simulink library "SCR"  (R2024b)
settings: Solver=VariableStepAuto  StartTime=0.0  StopTime=10.0  RelTol=1e-3
libraries: nesl_utility x29, fl_lib x26, sm_lib x16, ee_lib x7, slpidlib x4
(part 1 of 2)
settings Model: Creator=Michael  LastModifiedBy=Michael

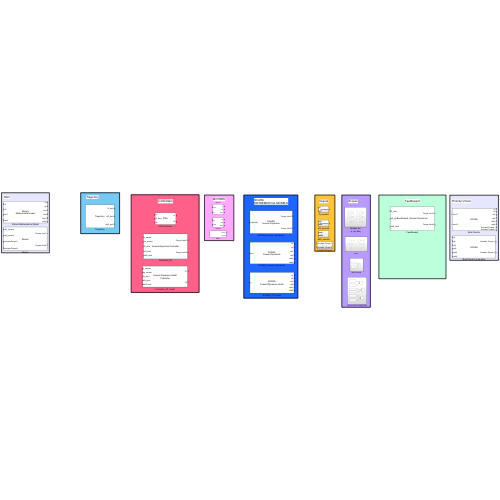
[thumbnail: Simulink's stored preview of the top-level diagram]
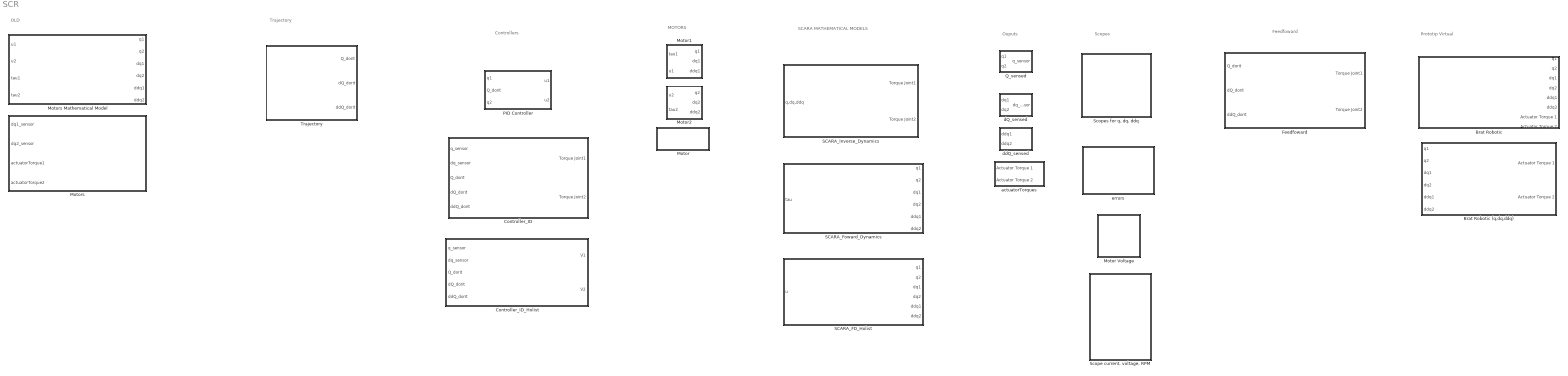
== system SCR ==
  note: MOTORS
  note: SCARA
      | MATHEMATICAL MODELS
  note: Scopes
  note: Ouputs
  note: Trajectory
  note: Controllers
  note: Feedfoward
  note: OLD
  note: Prototip Virtual
  Brat Robotic : Subsystem
      mask Display: disp("SCARA")
  Brat Robotic (q,dq,ddq) : Subsystem
      mask Display: disp("SCARA")
  Controller_ID : Subsystem
      mask Display: disp("Inverse Dynamics Controller")
  Controller_ID_Holist : Subsystem
      mask Display:
      | disp("Inverse Dynamics Holist\n")
      | disp("\nController")
  Feedfoward : Subsystem
      mask Display: disp("Feedfoward (Inverse Dynamics)")
  Motor : Subsystem
  Motor Voltage : Subsystem
  Motor1 : Subsystem
  Motor2 : Subsystem
  Motors : Subsystem
      mask Display: disp("Motors")
  Motors Mathematical Model : Subsystem
      mask Display:
      | disp("Motors\n")
      | disp("\nMathematical model")
  PID Controller : Subsystem
      mask Display: disp("PIDs")
  Q_sensed : Subsystem
  SCARA_FD_Holist : Subsystem
      mask Display:
      | disp("SCARA\n")
      | disp("\nFoward Dynamics Holist")
  SCARA_Foward_Dynamics : Subsystem
      mask Display:
      | disp("SCARA\n")
      | disp("\nFoward Dynamics")
  SCARA_Inverse_Dynamics : Subsystem
      mask Display:
      | disp("SCARA\n")
      | disp("\nInverse Dynamics")
  "Scope current, voltage, RPM" : Subsystem
  "Scopes for q, dq, ddq" : Subsystem
  Trajectory : Subsystem
      mask Display: disp("Trajectory")
  actuatorTorques : Subsystem
  dQ_sensed : Subsystem
  ddQ_sensed : Subsystem
  errors : Subsystem

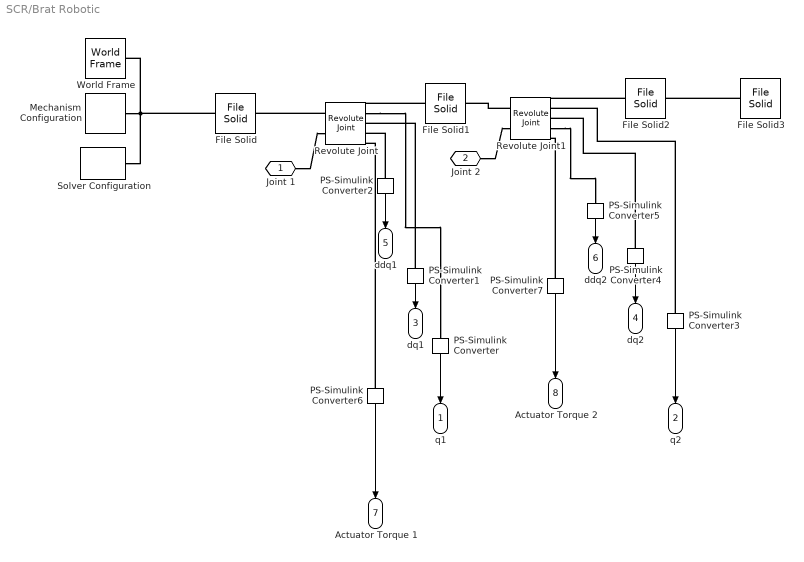
== system SCR/Brat Robotic ==
  File Solid : sm_lib/Body Elements/File Solid  ExtGeomFileName=C:\Users\Michael\Documents\Facultate\AN-IV\SCR\SCARA\robotCAD\baza.step  UnitType=FromFile  ExtGeomFileUnits=m  StepReaderType=HEX  ExportConvexHullGeometry=off  InertiaType=CalculateFromGeometry  BasedOnType=Density  Density=2700  DensityUnits=kg/m^3  Mass=1  MassUnits=kg  CenterOfMass=[0 0 0]  CenterOfMassUnits=m  MomentsOfInertia=[1 1 1]  MomentsOfInertiaUnits=kg*m^2  ProductsOfInertia=[0 0 0]  ProductsOfInertiaUnits=kg*m^2  GraphicType=FromGeometry  MarkerShape=Sphere  MarkerSize=10  GraphicVisPropType=SimpleVisualProperties  GraphicDiffuseColor=[0.5 0.5 0.5]  GraphicOpacity=1  GraphicSpecularColor=[0.5 0.5 0.5 1.0]  GraphicAmbientColor=[0.15 0.15 0.15 1.0]  GraphicEmissiveColor=[0.0 0.0 0.0 1.0]  GraphicShininess=75  DoExposeReferenceFrame=on  SerializedFrames=<Frames><Frame><Id>Frame1</Id><Value><Name>F1</Name><Origin><Source>GeometricFeature</Source><FeatureName>planar surface 2</FeatureName></Origin><PrimaryAxis><DefinedDirection>+Z</DefinedDirection><Source>ReferenceFrame</Source><SourceDirection>+Z</SourceDirection><FeatureName></FeatureName></PrimaryAxis><SecondaryAxis><DefinedDirection>+X</DefinedDirection><Source>ReferenceFrame</Source><SourceDirection>+X</SourceDirection><FeatureName></FeatureName></SecondaryAxis></Value></Frame></Frames>
  File Solid1 : sm_lib/Body Elements/File Solid  ExtGeomFileName=C:\Users\Michael\Documents\Facultate\AN-IV\SCR\SCARA\robotCAD\link1.step  UnitType=FromFile  ExtGeomFileUnits=m  StepReaderType=HEX  ExportConvexHullGeometry=off  InertiaType=CalculateFromGeometry  BasedOnType=Density  Density=2700  DensityUnits=kg/m^3  Mass=1  MassUnits=kg  CenterOfMass=[0 0 0]  CenterOfMassUnits=m  MomentsOfInertia=[1 1 1]  MomentsOfInertiaUnits=kg*m^2  ProductsOfInertia=[0 0 0]  ProductsOfInertiaUnits=kg*m^2  GraphicType=FromGeometry  MarkerShape=Sphere  MarkerSize=10  GraphicVisPropType=SimpleVisualProperties  GraphicDiffuseColor=[0.5 0.5 0.5]  GraphicOpacity=1  GraphicSpecularColor=[0.5 0.5 0.5 1.0]  GraphicAmbientColor=[0.15 0.15 0.15 1.0]  GraphicEmissiveColor=[0.0 0.0 0.0 1.0]  GraphicShininess=75  DoExposeReferenceFrame=on  SerializedFrames=<Frames><Frame><Id>Frame1</Id><Value><Name>F1</Name><Origin><Source>GeometricFeature</Source><FeatureName>circular curve 1</FeatureName></Origin><PrimaryAxis><DefinedDirection>+Z</DefinedDirection><Source>ReferenceFrame</Source><SourceDirection>+Z</SourceDirection><FeatureName></FeatureName></PrimaryAxis><SecondaryAxis><DefinedDirection>+X</DefinedDirection><Source>ReferenceFrame</Source><SourceDirection>+X</SourceDirection><FeatureName></FeatureName></SecondaryAxis></Value></Frame></Frames>
  File Solid2 : sm_lib/Body Elements/File Solid  ExtGeomFileName=C:\Users\Michael\Documents\Facultate\AN-IV\SCR\SCARA\robotCAD\link2.step  UnitType=FromFile  ExtGeomFileUnits=m  StepReaderType=HEX  ExportConvexHullGeometry=off  InertiaType=CalculateFromGeometry  BasedOnType=Density  Density=2700  DensityUnits=kg/m^3  Mass=1  MassUnits=kg  CenterOfMass=[0 0 0]  CenterOfMassUnits=m  MomentsOfInertia=[1 1 1]  MomentsOfInertiaUnits=kg*m^2  ProductsOfInertia=[0 0 0]  ProductsOfInertiaUnits=kg*m^2  GraphicType=FromGeometry  MarkerShape=Sphere  MarkerSize=10  GraphicVisPropType=SimpleVisualProperties  GraphicDiffuseColor=[0.5 0.5 0.5]  GraphicOpacity=1  GraphicSpecularColor=[0.5 0.5 0.5 1.0]  GraphicAmbientColor=[0.15 0.15 0.15 1.0]  GraphicEmissiveColor=[0.0 0.0 0.0 1.0]  GraphicShininess=75  DoExposeReferenceFrame=on  SerializedFrames=<Frames><Frame><Id>Frame1</Id><Value><Name>F1</Name><Origin><Source>GeometricFeature</Source><FeatureName>circular curve 1</FeatureName></Origin><PrimaryAxis><DefinedDirection>+Z</DefinedDirection><Source>ReferenceFrame</Source><SourceDirection>+Z</SourceDirection><FeatureName></FeatureName></PrimaryAxis><SecondaryAxis><DefinedDirection>+X</DefinedDirection><Source>ReferenceFrame</Source><SourceDirection>+X</SourceDirection><FeatureName></FeatureName></SecondaryAxis></Value></Frame></Frames>
  File Solid3 : sm_lib/Body Elements/File Solid  ExtGeomFileName=C:\Users\Michael\Documents\Facultate\AN-IV\SCR\SCARA\robotCAD\efector.step  UnitType=FromFile  ExtGeomFileUnits=m  StepReaderType=HEX  ExportConvexHullGeometry=off  InertiaType=CalculateFromGeometry  BasedOnType=Density  Density=2700  DensityUnits=kg/m^3  Mass=1  MassUnits=kg  CenterOfMass=[0 0 0]  CenterOfMassUnits=m  MomentsOfInertia=[1 1 1]  MomentsOfInertiaUnits=kg*m^2  ProductsOfInertia=[0 0 0]  ProductsOfInertiaUnits=kg*m^2  GraphicType=FromGeometry  MarkerShape=Sphere  MarkerSize=10  GraphicVisPropType=SimpleVisualProperties  GraphicDiffuseColor=[0.5 0.5 0.5]  GraphicOpacity=1  GraphicSpecularColor=[0.5 0.5 0.5 1.0]  GraphicAmbientColor=[0.15 0.15 0.15 1.0]  GraphicEmissiveColor=[0.0 0.0 0.0 1.0]  GraphicShininess=75  DoExposeReferenceFrame=off  SerializedFrames=<Frames><Frame><Id>Frame1</Id><Value><Name>F1</Name><Origin><Source>GeometricFeature</Source><FeatureName>planar surface 1</FeatureName></Origin><PrimaryAxis><DefinedDirection>+Z</DefinedDirection><Source>ReferenceFrame</Source><SourceDirection>+Z</SourceDirection><FeatureName></FeatureName></PrimaryAxis><SecondaryAxis><DefinedDirection>+X</DefinedDirection><Source>ReferenceFrame</Source><SourceDirection>+X</SourceDirection><FeatureName></FeatureName></SecondaryAxis></Value></Frame></Frames>
  Mechanism Configuration : sm_lib/Utilities/Mechanism Configuration  UniformGravity=Constant  GravityVector=[0 0 -9.80665]  GravityVectorUnits=m/s^2  LinearizationDelta=0.001  JointModeTransitionNonlinearIterations=2
  PS-Simulink Converter{,2..3,5..7} (6 alike) : nesl_utility/PS-Simulink Converter  PhysicalDomain=network_engine_domain  SubClassName=ps_output  LeftPortType=input  RightPortType=output  PseudoPeriodic=off  Frequencies=[]  VectorFormat=inherit  Unit=inherit  AffineConversion=off
  PS-Simulink Converter1 : nesl_utility/PS-Simulink Converter  PhysicalDomain=network_engine_domain  SubClassName=ps_output  LeftPortType=input  RightPortType=output  PseudoPeriodic=off  Frequencies=[]  VectorFormat=inherit  Unit=rad/s  AffineConversion=off
  PS-Simulink Converter4 : nesl_utility/PS-Simulink Converter  PhysicalDomain=network_engine_domain  SubClassName=ps_output  LeftPortType=input  RightPortType=output  PseudoPeriodic=off  Frequencies=[]  VectorFormat=inherit  Unit=rad/s  AffineConversion=off
  Revolute Joint : sm_lib/Joints/Revolute Joint  JointMode=Normal  CompositeWrenchDir=FollowerOnBase  CompositeWrenchFrame=BaseFrame  SenseConstraintForce=off  SenseConstraintTorque=off  SenseTotalForce=off  SenseTotalTorque=off  PositionTargetSpecify=off  PositionTargetPriority=High  PositionTargetValue=0  PositionTargetValueUnits=deg  VelocityTargetSpecify=off  VelocityTargetPriority=High  VelocityTargetValue=0  VelocityTargetValueUnits=deg/s  EquilibriumPosition=0  EquilibriumPositionUnits=deg  SpringStiffness=0  SpringStiffnessUnits=N*m/deg  DampingCoefficient=0  DampingCoefficientUnits=N*m/(deg/s)  LowerLimitSpecify=off  LowerLimitBound=-90  LowerLimitBoundUnits=deg  LowerLimitStiffness=1e4  LowerLimitStiffnessUnits=N*m/deg  LowerLimitDamping=10  LowerLimitDampingUnits=N*m/(deg/s)  LowerLimitTransitionRegionWidth=0.1  LowerLimitTransitionRegionWidthUnits=deg  UpperLimitSpecify=off  UpperLimitBound=90  UpperLimitBoundUnits=deg  UpperLimitStiffness=1e4  UpperLimitStiffnessUnits=N*m/deg  UpperLimitDamping=10  UpperLimitDampingUnits=N*m/(deg/s)  UpperLimitTransitionRegionWidth=0.1  UpperLimitTransitionRegionWidthUnits=deg  TorqueActuationMode=InputTorque  MotionActuationMode=ComputedMotion  SensePosition=on  SenseVelocity=on  SenseAcceleration=on  SenseTorqueForce=on  SenseLowerLimitTorqueForce=off  SenseUpperLimitTorqueForce=off
  Revolute Joint1 : sm_lib/Joints/Revolute Joint  JointMode=Normal  CompositeWrenchDir=FollowerOnBase  CompositeWrenchFrame=BaseFrame  SenseConstraintForce=off  SenseConstraintTorque=off  SenseTotalForce=off  SenseTotalTorque=off  PositionTargetSpecify=off  PositionTargetPriority=High  PositionTargetValue=0  PositionTargetValueUnits=deg  VelocityTargetSpecify=off  VelocityTargetPriority=High  VelocityTargetValue=0  VelocityTargetValueUnits=deg/s  EquilibriumPosition=0  EquilibriumPositionUnits=deg  SpringStiffness=0  SpringStiffnessUnits=N*m/deg  DampingCoefficient=0  DampingCoefficientUnits=N*m/(deg/s)  LowerLimitSpecify=off  LowerLimitBound=-90  LowerLimitBoundUnits=deg  LowerLimitStiffness=1e4  LowerLimitStiffnessUnits=N*m/deg  LowerLimitDamping=10  LowerLimitDampingUnits=N*m/(deg/s)  LowerLimitTransitionRegionWidth=0.1  LowerLimitTransitionRegionWidthUnits=deg  UpperLimitSpecify=off  UpperLimitBound=90  UpperLimitBoundUnits=deg  UpperLimitStiffness=1e4  UpperLimitStiffnessUnits=N*m/deg  UpperLimitDamping=10  UpperLimitDampingUnits=N*m/(deg/s)  UpperLimitTransitionRegionWidth=0.1  UpperLimitTransitionRegionWidthUnits=deg  TorqueActuationMode=InputTorque  MotionActuationMode=ComputedMotion  SensePosition=on  SenseVelocity=on  SenseAcceleration=on  SenseTorqueForce=on  SenseLowerLimitTorqueForce=off  SenseUpperLimitTorqueForce=off
  Solver Configuration : nesl_utility/Solver Configuration  PhysicalDomain=network_engine_domain  SubClassName=solver  LeftPortType=input  RightPortType=generic  Tones=[]  Harmonics=[]  SimulateNoise=off  Profile=off  UseLocalSampling=off  EnableSwitchedLinearOptims=on  FrequencyDomain=off  UseCCode=off  RelTol=0.001  AbsTol=0.001  MinStep=1e-09  ToWorkspace=off  RevertToSquareIcSolve=off  NumHomotopyIterations=100  PhasorMode=off  PhasorModeNumHarmonics=1  ConsistencySolver=NEWTON_XTOL_AFTER_FTOL  IndexReductionMethod=DerivativeReplacement  DoDC=off  ResidualTolerance=1e-09  ConsistencyTolSource=GLOBAL  ConsistencyAbsTol=0.001  ConsistencyRelTol=0.001  ConsistencyTolFactor=0.001  UseLocalSolver=off  LocalSolverChoice=NE_BACKWARD_EULER_ADVANCER  ResolveIndetEquations=on  FunctionEvalNumThread=1  LocalSolverSampleTime=0.001  DoFixedCost=off  MaxNonlinIter=3  MaxModeIter=2  ComputeImpulses=off  ImpulseIterations=2  LinearAlgebra=auto  LinearAlgebraNumThread=0  EquationFormulation=NE_TIME_EF  DelaysMemoryBudget=1024  AutomaticFiltering=on  FilteringTimeConstant=0.001  PartitionStorageMethod=AS_NEEDED  PartitionMemoryBudget=1024  PartitionMethod=ROBUST  MultibodyUseLocalSolver=off  MultibodyLocalSolverChoice=ODE1  MultibodyLocalSolverSampleTime=0.001
  World Frame : sm_lib/Frames and Transforms/World Frame
  Joint 1 : PMIOPort  Side=Left
  Joint 2 : PMIOPort  Port=2  Side=Left
  q1 : Outport
  q2 : Outport  Port=2
  dq1 : Outport  Port=3
  dq2 : Outport  Port=4
  ddq1 : Outport  Port=5
  ddq2 : Outport  Port=6
  Actuator Torque 1 : Outport  Port=7
  Actuator Torque 2 : Outport  Port=8
  wires:
  PS-Simulink Converter2/1 -> ddq1/1
  PS-Simulink Converter1/1 -> dq1/1
  PS-Simulink Converter/1 -> q1/1
  PS-Simulink Converter5/1 -> ddq2/1
  PS-Simulink Converter4/1 -> dq2/1
  PS-Simulink Converter3/1 -> q2/1
  PS-Simulink Converter6/1 -> Actuator Torque 1/1
  PS-Simulink Converter7/1 -> Actuator Torque 2/1
  connections:
  File Solid/RConn1 -- Mechanism Configuration/RConn1 -- Solver Configuration/RConn1 -- World Frame/RConn1
  Revolute Joint/LConn1 -- File Solid/LConn1
  File Solid1/RConn1 -- Revolute Joint/RConn1
  Revolute Joint1/LConn1 -- File Solid1/LConn1
  File Solid2/RConn1 -- Revolute Joint1/RConn1
  File Solid3/LConn1 -- File Solid2/LConn1
  Joint 1/RConn1 -- Revolute Joint/LConn2
  Joint 2/RConn1 -- Revolute Joint1/LConn2
  Revolute Joint/RConn2 -- PS-Simulink Converter/LConn1
  PS-Simulink Converter1/LConn1 -- Revolute Joint/RConn3
  PS-Simulink Converter2/LConn1 -- Revolute Joint/RConn4
  Revolute Joint1/RConn4 -- PS-Simulink Converter5/LConn1
  PS-Simulink Converter4/LConn1 -- Revolute Joint1/RConn3
  PS-Simulink Converter3/LConn1 -- Revolute Joint1/RConn2
  PS-Simulink Converter6/LConn1 -- Revolute Joint/RConn5
  PS-Simulink Converter7/LConn1 -- Revolute Joint1/RConn5

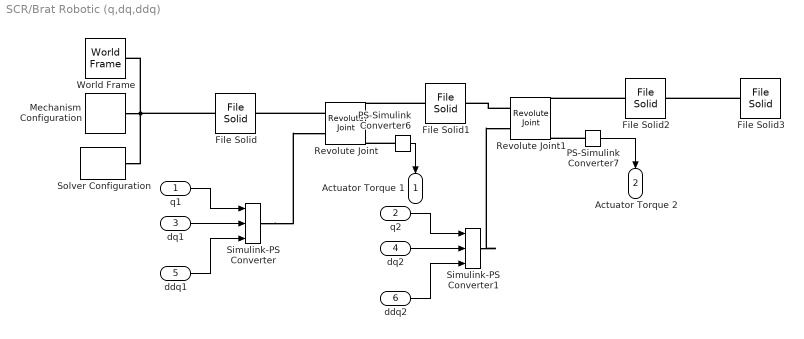
== system SCR/Brat Robotic (q,dq,ddq) ==
  q1 : Inport
  q2 : Inport  Port=2
  dq1 : Inport  Port=3
  dq2 : Inport  Port=4
  ddq1 : Inport  Port=5
  ddq2 : Inport  Port=6
  File Solid : sm_lib/Body Elements/File Solid  ExtGeomFileName=C:\Users\Michael\Documents\Facultate\AN-IV\SCR\SCARA\robotCAD\baza.step  UnitType=FromFile  ExtGeomFileUnits=m  StepReaderType=HEX  ExportConvexHullGeometry=off  InertiaType=CalculateFromGeometry  BasedOnType=Density  Density=2700  DensityUnits=kg/m^3  Mass=1  MassUnits=kg  CenterOfMass=[0 0 0]  CenterOfMassUnits=m  MomentsOfInertia=[1 1 1]  MomentsOfInertiaUnits=kg*m^2  ProductsOfInertia=[0 0 0]  ProductsOfInertiaUnits=kg*m^2  GraphicType=FromGeometry  MarkerShape=Sphere  MarkerSize=10  GraphicVisPropType=SimpleVisualProperties  GraphicDiffuseColor=[0.5 0.5 0.5]  GraphicOpacity=1  GraphicSpecularColor=[0.5 0.5 0.5 1.0]  GraphicAmbientColor=[0.15 0.15 0.15 1.0]  GraphicEmissiveColor=[0.0 0.0 0.0 1.0]  GraphicShininess=75  DoExposeReferenceFrame=on  SerializedFrames=<Frames><Frame><Id>Frame1</Id><Value><Name>F1</Name><Origin><Source>GeometricFeature</Source><FeatureName>planar surface 2</FeatureName></Origin><PrimaryAxis><DefinedDirection>+Z</DefinedDirection><Source>ReferenceFrame</Source><SourceDirection>+Z</SourceDirection><FeatureName></FeatureName></PrimaryAxis><SecondaryAxis><DefinedDirection>+X</DefinedDirection><Source>ReferenceFrame</Source><SourceDirection>+X</SourceDirection><FeatureName></FeatureName></SecondaryAxis></Value></Frame></Frames>
  File Solid1 : sm_lib/Body Elements/File Solid  ExtGeomFileName=C:\Users\Michael\Documents\Facultate\AN-IV\SCR\SCARA\robotCAD\link1.step  UnitType=FromFile  ExtGeomFileUnits=m  StepReaderType=HEX  ExportConvexHullGeometry=off  InertiaType=CalculateFromGeometry  BasedOnType=Density  Density=2700  DensityUnits=kg/m^3  Mass=1  MassUnits=kg  CenterOfMass=[0 0 0]  CenterOfMassUnits=m  MomentsOfInertia=[1 1 1]  MomentsOfInertiaUnits=kg*m^2  ProductsOfInertia=[0 0 0]  ProductsOfInertiaUnits=kg*m^2  GraphicType=FromGeometry  MarkerShape=Sphere  MarkerSize=10  GraphicVisPropType=SimpleVisualProperties  GraphicDiffuseColor=[0.5 0.5 0.5]  GraphicOpacity=1  GraphicSpecularColor=[0.5 0.5 0.5 1.0]  GraphicAmbientColor=[0.15 0.15 0.15 1.0]  GraphicEmissiveColor=[0.0 0.0 0.0 1.0]  GraphicShininess=75  DoExposeReferenceFrame=on  SerializedFrames=<Frames><Frame><Id>Frame1</Id><Value><Name>F1</Name><Origin><Source>GeometricFeature</Source><FeatureName>circular curve 1</FeatureName></Origin><PrimaryAxis><DefinedDirection>+Z</DefinedDirection><Source>ReferenceFrame</Source><SourceDirection>+Z</SourceDirection><FeatureName></FeatureName></PrimaryAxis><SecondaryAxis><DefinedDirection>+X</DefinedDirection><Source>ReferenceFrame</Source><SourceDirection>+X</SourceDirection><FeatureName></FeatureName></SecondaryAxis></Value></Frame></Frames>
  File Solid2 : sm_lib/Body Elements/File Solid  ExtGeomFileName=C:\Users\Michael\Documents\Facultate\AN-IV\SCR\SCARA\robotCAD\link2.step  UnitType=FromFile  ExtGeomFileUnits=m  StepReaderType=HEX  ExportConvexHullGeometry=off  InertiaType=CalculateFromGeometry  BasedOnType=Density  Density=2700  DensityUnits=kg/m^3  Mass=1  MassUnits=kg  CenterOfMass=[0 0 0]  CenterOfMassUnits=m  MomentsOfInertia=[1 1 1]  MomentsOfInertiaUnits=kg*m^2  ProductsOfInertia=[0 0 0]  ProductsOfInertiaUnits=kg*m^2  GraphicType=FromGeometry  MarkerShape=Sphere  MarkerSize=10  GraphicVisPropType=SimpleVisualProperties  GraphicDiffuseColor=[0.5 0.5 0.5]  GraphicOpacity=1  GraphicSpecularColor=[0.5 0.5 0.5 1.0]  GraphicAmbientColor=[0.15 0.15 0.15 1.0]  GraphicEmissiveColor=[0.0 0.0 0.0 1.0]  GraphicShininess=75  DoExposeReferenceFrame=on  SerializedFrames=<Frames><Frame><Id>Frame1</Id><Value><Name>F1</Name><Origin><Source>GeometricFeature</Source><FeatureName>circular curve 1</FeatureName></Origin><PrimaryAxis><DefinedDirection>+Z</DefinedDirection><Source>ReferenceFrame</Source><SourceDirection>+Z</SourceDirection><FeatureName></FeatureName></PrimaryAxis><SecondaryAxis><DefinedDirection>+X</DefinedDirection><Source>ReferenceFrame</Source><SourceDirection>+X</SourceDirection><FeatureName></FeatureName></SecondaryAxis></Value></Frame></Frames>
  File Solid3 : sm_lib/Body Elements/File Solid  ExtGeomFileName=C:\Users\Michael\Documents\Facultate\AN-IV\SCR\SCARA\robotCAD\efector.step  UnitType=FromFile  ExtGeomFileUnits=m  StepReaderType=HEX  ExportConvexHullGeometry=off  InertiaType=CalculateFromGeometry  BasedOnType=Density  Density=2700  DensityUnits=kg/m^3  Mass=1  MassUnits=kg  CenterOfMass=[0 0 0]  CenterOfMassUnits=m  MomentsOfInertia=[1 1 1]  MomentsOfInertiaUnits=kg*m^2  ProductsOfInertia=[0 0 0]  ProductsOfInertiaUnits=kg*m^2  GraphicType=FromGeometry  MarkerShape=Sphere  MarkerSize=10  GraphicVisPropType=SimpleVisualProperties  GraphicDiffuseColor=[0.5 0.5 0.5]  GraphicOpacity=1  GraphicSpecularColor=[0.5 0.5 0.5 1.0]  GraphicAmbientColor=[0.15 0.15 0.15 1.0]  GraphicEmissiveColor=[0.0 0.0 0.0 1.0]  GraphicShininess=75  DoExposeReferenceFrame=off  SerializedFrames=<Frames><Frame><Id>Frame1</Id><Value><Name>F1</Name><Origin><Source>GeometricFeature</Source><FeatureName>planar surface 1</FeatureName></Origin><PrimaryAxis><DefinedDirection>+Z</DefinedDirection><Source>ReferenceFrame</Source><SourceDirection>+Z</SourceDirection><FeatureName></FeatureName></PrimaryAxis><SecondaryAxis><DefinedDirection>+X</DefinedDirection><Source>ReferenceFrame</Source><SourceDirection>+X</SourceDirection><FeatureName></FeatureName></SecondaryAxis></Value></Frame></Frames>
  Mechanism Configuration : sm_lib/Utilities/Mechanism Configuration  UniformGravity=Constant  GravityVector=[0 0 -9.80665]  GravityVectorUnits=m/s^2  LinearizationDelta=0.001  JointModeTransitionNonlinearIterations=2
  PS-Simulink Converter6 : nesl_utility/PS-Simulink Converter  PhysicalDomain=network_engine_domain  SubClassName=ps_output  LeftPortType=input  RightPortType=output  PseudoPeriodic=off  Frequencies=[]  VectorFormat=inherit  Unit=inherit  AffineConversion=off
  PS-Simulink Converter7 : nesl_utility/PS-Simulink Converter  PhysicalDomain=network_engine_domain  SubClassName=ps_output  LeftPortType=input  RightPortType=output  PseudoPeriodic=off  Frequencies=[]  VectorFormat=inherit  Unit=inherit  AffineConversion=off
  Revolute Joint : sm_lib/Joints/Revolute Joint  JointMode=Normal  CompositeWrenchDir=FollowerOnBase  CompositeWrenchFrame=BaseFrame  SenseConstraintForce=off  SenseConstraintTorque=off  SenseTotalForce=off  SenseTotalTorque=off  PositionTargetSpecify=off  PositionTargetPriority=High  PositionTargetValue=0  PositionTargetValueUnits=deg  VelocityTargetSpecify=off  VelocityTargetPriority=High  VelocityTargetValue=0  VelocityTargetValueUnits=deg/s  EquilibriumPosition=0  EquilibriumPositionUnits=deg  SpringStiffness=0  SpringStiffnessUnits=N*m/deg  DampingCoefficient=0  DampingCoefficientUnits=N*m/(deg/s)  LowerLimitSpecify=off  LowerLimitBound=-90  LowerLimitBoundUnits=deg  LowerLimitStiffness=1e4  LowerLimitStiffnessUnits=N*m/deg  LowerLimitDamping=10  LowerLimitDampingUnits=N*m/(deg/s)  LowerLimitTransitionRegionWidth=0.1  LowerLimitTransitionRegionWidthUnits=deg  UpperLimitSpecify=off  UpperLimitBound=90  UpperLimitBoundUnits=deg  UpperLimitStiffness=1e4  UpperLimitStiffnessUnits=N*m/deg  UpperLimitDamping=10  UpperLimitDampingUnits=N*m/(deg/s)  UpperLimitTransitionRegionWidth=0.1  UpperLimitTransitionRegionWidthUnits=deg  TorqueActuationMode=ComputedTorque  MotionActuationMode=InputMotion  SensePosition=on  SenseVelocity=on  SenseAcceleration=on  SenseTorqueForce=on  SenseLowerLimitTorqueForce=off  SenseUpperLimitTorqueForce=off
  Revolute Joint1 : sm_lib/Joints/Revolute Joint  JointMode=Normal  CompositeWrenchDir=FollowerOnBase  CompositeWrenchFrame=BaseFrame  SenseConstraintForce=off  SenseConstraintTorque=off  SenseTotalForce=off  SenseTotalTorque=off  PositionTargetSpecify=off  PositionTargetPriority=High  PositionTargetValue=0  PositionTargetValueUnits=deg  VelocityTargetSpecify=off  VelocityTargetPriority=High  VelocityTargetValue=0  VelocityTargetValueUnits=deg/s  EquilibriumPosition=0  EquilibriumPositionUnits=deg  SpringStiffness=0  SpringStiffnessUnits=N*m/deg  DampingCoefficient=0  DampingCoefficientUnits=N*m/(deg/s)  LowerLimitSpecify=off  LowerLimitBound=-90  LowerLimitBoundUnits=deg  LowerLimitStiffness=1e4  LowerLimitStiffnessUnits=N*m/deg  LowerLimitDamping=10  LowerLimitDampingUnits=N*m/(deg/s)  LowerLimitTransitionRegionWidth=0.1  LowerLimitTransitionRegionWidthUnits=deg  UpperLimitSpecify=off  UpperLimitBound=90  UpperLimitBoundUnits=deg  UpperLimitStiffness=1e4  UpperLimitStiffnessUnits=N*m/deg  UpperLimitDamping=10  UpperLimitDampingUnits=N*m/(deg/s)  UpperLimitTransitionRegionWidth=0.1  UpperLimitTransitionRegionWidthUnits=deg  TorqueActuationMode=InputTorque  MotionActuationMode=ComputedMotion  SensePosition=on  SenseVelocity=on  SenseAcceleration=on  SenseTorqueForce=on  SenseLowerLimitTorqueForce=off  SenseUpperLimitTorqueForce=off
  Simulink-PS Converter : nesl_utility/Simulink-PS Converter  PhysicalDomain=network_engine_domain  SubClassName=ps_input  LeftPortType=input  RightPortType=output  PseudoPeriodic=off  Frequencies=[]  NoiseDistribution=none  NoiseParameters=[]  Unit=1  AffineConversion=off  FilteringAndDerivatives=provide  SimscapeFilterOrder=1  InputFilterTimeConstant=0.001  UdotUserProvided=2
  Simulink-PS Converter1 : nesl_utility/Simulink-PS Converter  PhysicalDomain=network_engine_domain  SubClassName=ps_input  LeftPortType=input  RightPortType=output  PseudoPeriodic=off  Frequencies=[]  NoiseDistribution=none  NoiseParameters=[]  Unit=1  AffineConversion=off  FilteringAndDerivatives=provide  SimscapeFilterOrder=1  InputFilterTimeConstant=0.001  UdotUserProvided=2
  Solver Configuration : nesl_utility/Solver Configuration  PhysicalDomain=network_engine_domain  SubClassName=solver  LeftPortType=input  RightPortType=generic  Tones=[]  Harmonics=[]  SimulateNoise=off  Profile=off  UseLocalSampling=off  EnableSwitchedLinearOptims=on  FrequencyDomain=off  UseCCode=off  RelTol=0.001  AbsTol=0.001  MinStep=1e-09  ToWorkspace=off  RevertToSquareIcSolve=off  NumHomotopyIterations=100  PhasorMode=off  PhasorModeNumHarmonics=1  ConsistencySolver=NEWTON_XTOL_AFTER_FTOL  IndexReductionMethod=DerivativeReplacement  DoDC=off  ResidualTolerance=1e-09  ConsistencyTolSource=GLOBAL  ConsistencyAbsTol=0.001  ConsistencyRelTol=0.001  ConsistencyTolFactor=0.001  UseLocalSolver=off  LocalSolverChoice=NE_BACKWARD_EULER_ADVANCER  ResolveIndetEquations=on  FunctionEvalNumThread=1  LocalSolverSampleTime=0.001  DoFixedCost=off  MaxNonlinIter=3  MaxModeIter=2  ComputeImpulses=off  ImpulseIterations=2  LinearAlgebra=auto  LinearAlgebraNumThread=0  EquationFormulation=NE_TIME_EF  DelaysMemoryBudget=1024  AutomaticFiltering=on  FilteringTimeConstant=0.001  PartitionStorageMethod=AS_NEEDED  PartitionMemoryBudget=1024  PartitionMethod=ROBUST  MultibodyUseLocalSolver=off  MultibodyLocalSolverChoice=ODE1  MultibodyLocalSolverSampleTime=0.001
  World Frame : sm_lib/Frames and Transforms/World Frame
  Actuator Torque 1 : Outport
  Actuator Torque 2 : Outport  Port=2
  wires:
  PS-Simulink Converter6/1 -> Actuator Torque 1/1
  PS-Simulink Converter7/1 -> Actuator Torque 2/1
  q1/1 -> Simulink-PS Converter/1
  dq1/1 -> Simulink-PS Converter/2
  ddq1/1 -> Simulink-PS Converter/3
  dq2/1 -> Simulink-PS Converter1/2
  q2/1 -> Simulink-PS Converter1/1
  ddq2/1 -> Simulink-PS Converter1/3
  connections:
  File Solid/RConn1 -- Mechanism Configuration/RConn1 -- Solver Configuration/RConn1 -- World Frame/RConn1
  Revolute Joint/LConn1 -- File Solid/LConn1
  File Solid1/RConn1 -- Revolute Joint/RConn1
  Revolute Joint1/LConn1 -- File Solid1/LConn1
  File Solid2/RConn1 -- Revolute Joint1/RConn1
  File Solid3/LConn1 -- File Solid2/LConn1
  PS-Simulink Converter6/LConn1 -- Revolute Joint/RConn5
  PS-Simulink Converter7/LConn1 -- Revolute Joint1/RConn5
  Simulink-PS Converter/RConn1 -- Revolute Joint/LConn2
  Simulink-PS Converter1/RConn1 -- Revolute Joint1/LConn2

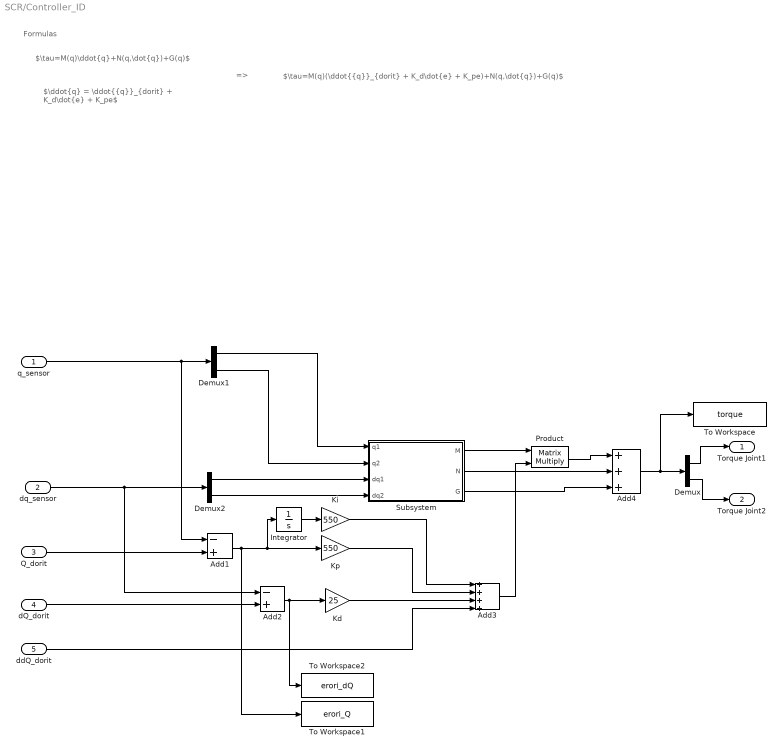
== system SCR/Controller_ID ==
  note: Formulas
  note: $\ddot{q} = \ddot{{q}}_{dorit} + K_d\dot{e} + K_pe$
  note: =>
  note: $\tau=M(q)\ddot{q}​+N(q,\dot{q})+G(q)$
  note: $\tau=M(q)(\ddot{{q}}_{dorit} + K_d\dot{e} + K_pe​)+N(q,\dot{q})+G(q)$
  q_sensor : Inport
  dq_sensor : Inport  Port=2
  Q_dorit : Inport  Port=3
  dQ_dorit : Inport  Port=4
  ddQ_dorit : Inport  Port=5
  Add1 : Sum  Inputs=-+
  Add2 : Sum  Inputs=-+
  Add3 : Sum  Inputs=++++
  Add4 : Sum  Inputs=+++
  Demux : Demux  Outputs=2
  Demux1 : Demux  Outputs=2
  Demux2 : Demux  Outputs=2
  Integrator : Integrator
  Kd : Gain  Gain=25
  Ki : Gain  Gain=550
  Kp : Gain  Gain=550
  Product : Product  Multiplication=Matrix(*)
  Subsystem : Subsystem
      mask Display: disp("Tau Components")
  To Workspace : ToWorkspace  VariableName=torque  SaveFormat=Timeseries  SampleTime=-1
  To Workspace1 : ToWorkspace  VariableName=erori_Q  SaveFormat=Timeseries  SampleTime=-1
  To Workspace2 : ToWorkspace  VariableName=erori_dQ  SaveFormat=Timeseries  SampleTime=-1
  Torque Joint1 : Outport
  Torque Joint2 : Outport  Port=2
  wires:
  Demux1/2 -> Subsystem/2(q2)
  dQ_dorit/1 -> Add2/2
  Add1/1 -> Kp/1, Integrator/1, To Workspace1/1
  Add2/1 -> Kd/1, To Workspace2/1
  Add3/1 -> Product/2
  Add4/1 -> To Workspace/1, Demux/1
  Demux/2 -> Torque Joint2/1
  Demux/1 -> Torque Joint1/1
  Q_dorit/1 -> Add1/2
  q_sensor/1 -> Add1/1, Demux1/1
  dq_sensor/1 -> Add2/1, Demux2/1
  Subsystem/1(M) -> Product/1
  Demux2/1 -> Subsystem/3(dq1)
  Demux2/2 -> Subsystem/4(dq2)
  Subsystem/2(N) -> Add4/2
  Demux1/1 -> Subsystem/1(q1)
  ddQ_dorit/1 -> Add3/4
  Kd/1 -> Add3/3
  Kp/1 -> Add3/2
  Ki/1 -> Add3/1
  Integrator/1 -> Ki/1
  Subsystem/3(G) -> Add4/3
  Product/1 -> Add4/1

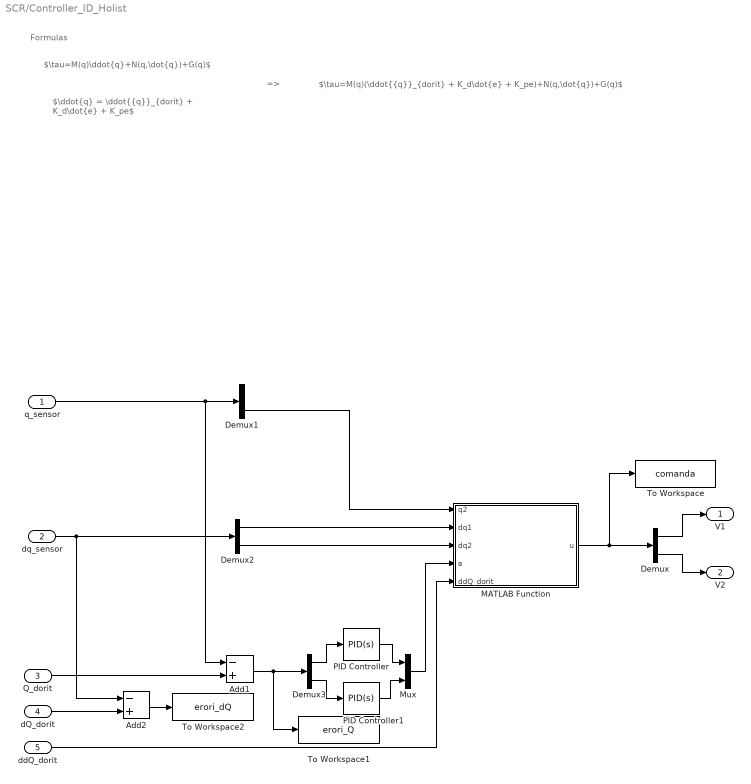
== system SCR/Controller_ID_Holist ==
  note: $\tau=M(q)(\ddot{{q}}_{dorit} + K_d\dot{e} + K_pe​)+N(q,\dot{q})+G(q)$
  note: $\tau=M(q)\ddot{q}​+N(q,\dot{q})+G(q)$
  note: =>
  note: $\ddot{q} = \ddot{{q}}_{dorit} + K_d\dot{e} + K_pe$
  note: Formulas
  q_sensor : Inport
  dq_sensor : Inport  Port=2
  Q_dorit : Inport  Port=3
  dQ_dorit : Inport  Port=4
  ddQ_dorit : Inport  Port=5
  Add1 : Sum  Inputs=-+
  Add2 : Sum  Inputs=-+
  Demux{,1..3} (4 alike) : Demux  Outputs=2
  MATLAB Function : MATLAB Function  TreatAsAtomicUnit=on
  Mux : Mux  Inputs=2
  PID Controller : slpidlib/PID Controller  Controller=PID  Form=Parallel  TimeDomain=Continuous-time  UseExternalTs=off  SampleTime=-1  IntegratorMethod=Forward Euler  FilterMethod=Forward Euler  ControllerParametersSource=internal  P=14.7787089689118  I=5.05842239486125  UseKiTs=off  D=9.92816544136059  UseExternalDerivativeSource=off  N=1142.8279760416  UseFilter=on  TunerSelectOption=Transfer Function Based (PID Tuner App)  InitialConditionSource=internal  InitialConditionForIntegrator=0  InitialConditionForFilter=0  DifferentiatorICPrevScaledInput=0  ExternalReset=none  TrackingMode=off  Kt=1  LimitOutput=off  SatLimitsSource=internal  UpperSaturationLimit=0  LowerSaturationLimit=0  LinearizeAsGain=on  AntiWindupMode=none  Kb=1  LimitIntegrator=off  UpperIntegratorSaturationLimit=inf  LowerIntegratorSaturationLimit=-inf  POutMin=[]  POutMax=[]  IOutMin=[]  IOutMax=[]  DOutMin=[]  DOutMax=[]  NOutMin=[]  NOutMax=[]  SumOutMin=[]  SumOutMax=[]  SaturationOutMin=[]  SaturationOutMax=[]  PParamMin=[]  PParamMax=[]  IParamMin=[]  IParamMax=[]  DParamMin=[]  DParamMax=[]  NParamMin=[]  NParamMax=[]  KbParamMin=[]  KbParamMax=[]  KtParamMin=[]  KtParamMax=[]  KbOutMin=[]  KbOutMax=[]  KtOutMin=[]  KtOutMax=[]  IntegratorOutMin=[]  IntegratorOutMax=[]  FilterOutMin=[]  FilterOutMax=[]  SumI1OutMin=[]  SumI1OutMax=[]  SumI2OutMin=[]  SumI2OutMax=[]  SumI3OutMin=[]  SumI3OutMax=[]  SumI4OutMin=[]  SumI4OutMax=[]  SumDOutMin=[]  SumDOutMax=[]  DifferentiatorOutMin=[]  DifferentiatorOutMax=[]  FilterDiffOutCoefMin=[]  FilterDiffOutCoefMax=[]  ReciprocalOutMin=[]  ReciprocalOutMax=[]  SumDenOutMin=[]  SumDenOutMax=[]  SumNumOutMin=[]  SumNumOutMax=[]  DivideOutMin=[]  DivideOutMax=[]  UdiffTsProdOutMin=[]  UdiffTsProdOutMax=[]  NTsProdOutMin=[]  NTsProdOutMax=[]  UintegralTsProdOutMin=[]  UintegralTsProdOutMax=[]  UngainTsProdOutMin=[]  UngainTsProdOutMax=[]  ClampingZeroOutDataTypeStr=Inherit: Inherit via back propagation  ClampingZeroOutMin=[]  ClampingZeroOutMax=[]  FilterDenConstantOutDataTypeStr=Inherit: Inherit via back propagation  FilterDenConstantOutMin=[]  FilterDenConstantOutMax=[]  PCopyOutDataTypeStr=Inherit: Inherit via back propagation  PCopyOutMin=[]  PCopyOutMax=[]  NCopyOutDataTypeStr=Inherit: Inherit via back propagation  NCopyOutMin=[]  NCopyOutMax=[]  IntegratorContinuousStateAttributes=''  IntegratorStateMustResolveToSignalObject=off  IntegratorRTWStateStorageClass=Auto  FilterContinuousStateAttributes=''  FilterStateMustResolveToSignalObject=off  FilterRTWStateStorageClass=Auto  ParallelPVariant=InternalParameters  IdealPVariant=Disabled  IVariant=InternalParameters  DVariant=InternalParameters  IntegratorVariant=Continuous  SatVariant=Disabled  AWVariant=Passthrough  PCopyVariant=Disabled  TRVariant=Disabled  FdbkBlocksVariant=Forward  IdealPFdbkVariant=Disabled  SatFdbkVariant=Disabled  DerivativeFilterVariant=ContFilter  NVariant=InternalParameters  NCopyVariant=Disabled  FilterICVariant=InternalICsFilter  IntegratorICVariant=InternalICs  ExternalResetVariant=Disabled  TRSumVariant=Passthrough  SumFdbkVariant=Disabled  SumVariant=Sum_PID  TsampFilterVariant=InternalTs  TsampNgainVariant=Passthrough  TsampIntegralVariant=Disabled_SignalSpec  ExternalSaturationOutDataTypeStr=Inherit: Same as second input  DerivativeSourceVariant=ErrorSignal  PreIntVariant=InternalPreInt
  PID Controller1 : slpidlib/PID Controller  Controller=PID  Form=Parallel  TimeDomain=Continuous-time  UseExternalTs=off  SampleTime=-1  IntegratorMethod=Forward Euler  FilterMethod=Forward Euler  ControllerParametersSource=internal  P=16.3330424592972  I=6.55014962380407  UseKiTs=off  D=9.91721708236017  UseExternalDerivativeSource=off  N=1142.8279760416  UseFilter=on  TunerSelectOption=Transfer Function Based (PID Tuner App)  InitialConditionSource=internal  InitialConditionForIntegrator=0  InitialConditionForFilter=0  DifferentiatorICPrevScaledInput=0  ExternalReset=none  TrackingMode=off  Kt=1  LimitOutput=off  SatLimitsSource=internal  UpperSaturationLimit=24  LowerSaturationLimit=-24  LinearizeAsGain=on  AntiWindupMode=none  Kb=1  LimitIntegrator=off  UpperIntegratorSaturationLimit=inf  LowerIntegratorSaturationLimit=-inf  POutMin=[]  POutMax=[]  IOutMin=[]  IOutMax=[]  DOutMin=[]  DOutMax=[]  NOutMin=[]  NOutMax=[]  SumOutMin=[]  SumOutMax=[]  SaturationOutMin=[]  SaturationOutMax=[]  PParamMin=[]  PParamMax=[]  IParamMin=[]  IParamMax=[]  DParamMin=[]  DParamMax=[]  NParamMin=[]  NParamMax=[]  KbParamMin=[]  KbParamMax=[]  KtParamMin=[]  KtParamMax=[]  KbOutMin=[]  KbOutMax=[]  KtOutMin=[]  KtOutMax=[]  IntegratorOutMin=[]  IntegratorOutMax=[]  FilterOutMin=[]  FilterOutMax=[]  SumI1OutMin=[]  SumI1OutMax=[]  SumI2OutMin=[]  SumI2OutMax=[]  SumI3OutMin=[]  SumI3OutMax=[]  SumI4OutMin=[]  SumI4OutMax=[]  SumDOutMin=[]  SumDOutMax=[]  DifferentiatorOutMin=[]  DifferentiatorOutMax=[]  FilterDiffOutCoefMin=[]  FilterDiffOutCoefMax=[]  ReciprocalOutMin=[]  ReciprocalOutMax=[]  SumDenOutMin=[]  SumDenOutMax=[]  SumNumOutMin=[]  SumNumOutMax=[]  DivideOutMin=[]  DivideOutMax=[]  UdiffTsProdOutMin=[]  UdiffTsProdOutMax=[]  NTsProdOutMin=[]  NTsProdOutMax=[]  UintegralTsProdOutMin=[]  UintegralTsProdOutMax=[]  UngainTsProdOutMin=[]  UngainTsProdOutMax=[]  ClampingZeroOutDataTypeStr=Inherit: Inherit via back propagation  ClampingZeroOutMin=[]  ClampingZeroOutMax=[]  FilterDenConstantOutDataTypeStr=Inherit: Inherit via back propagation  FilterDenConstantOutMin=[]  FilterDenConstantOutMax=[]  PCopyOutDataTypeStr=Inherit: Inherit via back propagation  PCopyOutMin=[]  PCopyOutMax=[]  NCopyOutDataTypeStr=Inherit: Inherit via back propagation  NCopyOutMin=[]  NCopyOutMax=[]  IntegratorContinuousStateAttributes=''  IntegratorStateMustResolveToSignalObject=off  IntegratorRTWStateStorageClass=Auto  FilterContinuousStateAttributes=''  FilterStateMustResolveToSignalObject=off  FilterRTWStateStorageClass=Auto  ParallelPVariant=InternalParameters  IdealPVariant=Disabled  IVariant=InternalParameters  DVariant=InternalParameters  IntegratorVariant=Continuous  SatVariant=Disabled  AWVariant=Passthrough  PCopyVariant=Disabled  TRVariant=Disabled  FdbkBlocksVariant=Forward  IdealPFdbkVariant=Disabled  SatFdbkVariant=Disabled  DerivativeFilterVariant=ContFilter  NVariant=InternalParameters  NCopyVariant=Disabled  FilterICVariant=InternalICsFilter  IntegratorICVariant=InternalICs  ExternalResetVariant=Disabled  TRSumVariant=Passthrough  SumFdbkVariant=Disabled  SumVariant=Sum_PID  TsampFilterVariant=InternalTs  TsampNgainVariant=Passthrough  TsampIntegralVariant=Disabled_SignalSpec  ExternalSaturationOutDataTypeStr=Inherit: Same as second input  DerivativeSourceVariant=ErrorSignal  PreIntVariant=InternalPreInt
  To Workspace : ToWorkspace  VariableName=comanda  SaveFormat=Timeseries  SampleTime=-1
  To Workspace1 : ToWorkspace  VariableName=erori_Q  SaveFormat=Timeseries  SampleTime=-1
  To Workspace2 : ToWorkspace  VariableName=erori_dQ  SaveFormat=Timeseries  SampleTime=-1
  V1 : Outport
  V2 : Outport  Port=2
  wires:
  Demux2/1 -> MATLAB Function/2(dq1)
  Demux1/2 -> MATLAB Function/1(q2)
  Mux/1 -> MATLAB Function/4(e)
  PID Controller1/1 -> Mux/2
  PID Controller/1 -> Mux/1
  Demux3/2 -> PID Controller1/1
  Demux3/1 -> PID Controller/1
  Add1/1 -> To Workspace1/1, Demux3/1
  MATLAB Function/1(u) -> To Workspace/1, Demux/1
  ddQ_dorit/1 -> MATLAB Function/5(ddQ_dorit)
  Demux2/2 -> MATLAB Function/3(dq2)
  dq_sensor/1 -> Add2/1, Demux2/1
  q_sensor/1 -> Demux1/1, Add1/1
  Q_dorit/1 -> Add1/2
  Demux/1 -> V1/1
  Demux/2 -> V2/1
  dQ_dorit/1 -> Add2/2
  Add2/1 -> To Workspace2/1

== system SCR/Feedfoward ==
  note: Formulas
  note: $\tau=M(q)\ddot{q}​+N(q,\dot{q})+G(q)$
  Q_dorit : Inport
  dQ_dorit : Inport  Port=2
  ddQ_dorit : Inport  Port=3
  Add4 : Sum  Inputs=+++
  Demux : Demux  Outputs=2
  Demux1 : Demux  Outputs=2
  Demux2 : Demux  Outputs=2
  Product : Product  Multiplication=Matrix(*)
  Subsystem : Subsystem
      mask Display: disp("Tau Components")
  Torque Joint1 : Outport
  Torque Joint2 : Outport  Port=2
  wires:
  Product/1 -> Add4/1
  Add4/1 -> Demux/1
  Demux/2 -> Torque Joint2/1
  Demux/1 -> Torque Joint1/1
  Subsystem/3(G) -> Add4/3
  Subsystem/1(M) -> Product/1
  Subsystem/2(N) -> Add4/2
  Q_dorit/1 -> Demux1/1
  Demux1/1 -> Subsystem/1(q1)
  Demux1/2 -> Subsystem/2(q2)
  dQ_dorit/1 -> Demux2/1
  Demux2/1 -> Subsystem/3(dq1)
  Demux2/2 -> Subsystem/4(dq2)
  ddQ_dorit/1 -> Product/2

== system SCR/Motor ==
  Controlled Voltage Source : fl_lib/Electrical/Electrical Sources/Controlled Voltage Source
  DC Motor : ee_lib/Electromechanical/Brushed Motors/DC Motor  field_option=ee.enum.field_option.pm  Rf=100 Ohm  Lf=1 H  Laf=0.15 H  If0=0 A  parameterization=ee.enum.dcparam_option.circuit_param  Ra=0.108 Ohm  La=0.0336 mH  emf_or_torque=ee.enum.emf_or_torque.ki  Kv=0.072e-3 V/rpm  Ki=15.6 m*mN/A  T_stall=0.24e-3 N*m  w_max=19100 rpm  w_rated=15000 rpm  P_rated=0.08 W  V_rated=1.5 V  lam_param=ee.enum.lam_param.current  i_noload=274 mA  V_i_noload=12 V  J=77.6 cm^2*g  lam=0 N*m*s/rad  speed0=0 rpm  t_fault_armature=1 s  t_fault_field=1 s  fault_action=simscape.enum.assert.action.none  alpha=3.93e-3 1/K  Tmeas=25 degC  thermal_mass=100 J/K  initial_temperature=25 degC
  Electrical Reference : fl_lib/Electrical/Electrical Elements/Electrical Reference
  Ideal Rotational Motion Sensor : fl_lib/Mechanical/Mechanical Sensors/Ideal Rotational Motion Sensor  reference=foundation.enum.MeasurementReference.difference  acceleration_port=false  velocity_port=true  position_port=true  wrap_angle=false  offset=0 rad
  Mechanical Rotational Reference : fl_lib/Mechanical/Rotational Elements/Mechanical Rotational Reference
  PS-Simulink Converter : nesl_utility/PS-Simulink Converter  PhysicalDomain=network_engine_domain  SubClassName=ps_output  LeftPortType=input  RightPortType=output  PseudoPeriodic=off  Frequencies=[]  VectorFormat=inherit  Unit=inherit  AffineConversion=off
  Scope : Scope
  Conn1 : PMIOPort  Side=Right
  Conn2 : PMIOPort  Port=2  Side=Right
  wires:
  PS-Simulink Converter/1 -> Scope/1
  connections:
  Controlled Voltage Source/LConn1 -- DC Motor/LConn1
  Controlled Voltage Source/RConn2 -- Electrical Reference/LConn1 -- DC Motor/RConn1
  Mechanical Rotational Reference/LConn1 -- Ideal Rotational Motion Sensor/RConn1 -- DC Motor/RConn2
  PS-Simulink Converter/LConn1 -- Ideal Rotational Motion Sensor/RConn2
  Ideal Rotational Motion Sensor/LConn1 -- DC Motor/LConn2
  Controlled Voltage Source/RConn1 -- Conn2/RConn1
  Ideal Rotational Motion Sensor/RConn3 -- Conn1/RConn1

== system SCR/Motor Voltage ==
  motorTorques : Scope  NumInputPorts=2
  wires:
  [u1] -> motorTorques/1
  [u2] -> motorTorques/2

== system SCR/Motor1 ==
  tau1 : Inport
  u1 : Inport  Port=2
  MATLAB Function : MATLAB Function  TreatAsAtomicUnit=on
  position : Integrator
  velocity : Integrator
  q1 : Outport
  dq1 : Outport  Port=2
  ddq1 : Outport  Port=3
  tag scope: ddq1=global, dq1=global, q1=global, u1=global
  wires:
  MATLAB Function/1(ddq) -> [ddq1], ddq1/1, velocity/1
  u1/1 -> [u1], MATLAB Function/2(u)
  tau1/1 -> MATLAB Function/1(tau)
  velocity/1 -> [dq1], dq1/1, MATLAB Function/3(dq), position/1
  position/1 -> [q1], q1/1

== system SCR/Motor2 ==
  u2 : Inport
  tau2 : Inport  Port=2
  MATLAB Function1 : MATLAB Function  TreatAsAtomicUnit=on
  position1 : Integrator
  velocity1 : Integrator
  q2 : Outport
  dq2 : Outport  Port=2
  ddq2 : Outport  Port=3
  tag scope: ddq2=global, dq2=global, q2=global
  wires:
  MATLAB Function1/1(ddq) -> [ddq2], ddq2/1, velocity1/1
  velocity1/1 -> [dq2], dq2/1, MATLAB Function1/3(dq), position1/1
  tau2/1 -> MATLAB Function1/1(tau)
  position1/1 -> [q2], q2/1
  u2/1 -> [u2], MATLAB Function1/2(u)

== system SCR/Motors ==
  note: Motorul nu este inca modelat complet, dar ar trebui sa fie destul. Ideal source torque-ul inmultit cu "-1" functioneaza ca un moment de rezistenta
  note: OLD SHIT
  note: Formulas
  note: $\omega = r\omega_{joint}$
  note: (revolute joint); N = gear ratio
  note: $\omega = N\omega_{joint}$
  note: where,
  note: $V = \frac{\tau}{k_{\tau}}R + k_E * \omega$
  note: (prismatic joint); r = displacement per revolution
  note: Formulas
  note: $V_{motor} = (q_{dorit} - q_{sensor}) * Kp + (\dot{q}_{dorit} - \dot{q}_{sensor}) * Kd$
  note: Asta e pentru feedfowardul cu inverse dynamics
  dq1_sensor : Inport
  dq2_sensor : Inport  Port=2
  actuatorTorque1 : Inport  Port=3
  actuatorTorque2 : Inport  Port=4
  Motor : Subsystem
      settings: PortSchema="{\"entries\":[{\"content\":{\"sides\":[{\"content\":{\"connectorIds\":[\"LConn1\"]},\"type\":\"ConnectorPlacement.EquallySpacedRectSide\",\"uuid\":\"39e40abe-083b-42cd-b401-a01d4246ad16\"},{\"content\":{\"connectorIds\":[\"In1\",\"RConn1\",\"In2\"],\"side\":\"RIGHT\"},\"type\":\"ConnectorPlacement.EquallySpacedRectSide\",\"uuid\":\"321e8228-06c3-42ae-935e-004b5db31bc2\"},{\"content\":{\"side\":\"TOP\"},\"type\":\"ConnectorPlacement.EquallySpacedRectSide\",\"uuid\":\"7a7ef2a1-3d21-46bd-9477-6821b2be4d0d\"}]},\"type\":\"ConnectorPlacement.EquallySpacedConnector\",\"uuid\":\"bceb85c7-25a5-44d0-bafc-eda31cc970da\"}],\"packageUris\":[\"http://schema.mathworks.com/mf0/Connector/R2020b\"],\"version\":\"1.0\"}"
      mask Display: disp("DC Motor")
  Motor1 : Subsystem
      settings: PortSchema="{\"entries\":[{\"content\":{\"sides\":[{\"content\":{\"connectorIds\":[\"LConn1\"]},\"type\":\"ConnectorPlacement.EquallySpacedRectSide\",\"uuid\":\"39e40abe-083b-42cd-b401-a01d4246ad16\"},{\"content\":{\"connectorIds\":[\"In1\",\"RConn1\",\"In2\"],\"side\":\"RIGHT\"},\"type\":\"ConnectorPlacement.EquallySpacedRectSide\",\"uuid\":\"321e8228-06c3-42ae-935e-004b5db31bc2\"},{\"content\":{\"side\":\"TOP\"},\"type\":\"ConnectorPlacement.EquallySpacedRectSide\",\"uuid\":\"7a7ef2a1-3d21-46bd-9477-6821b2be4d0d\"}]},\"type\":\"ConnectorPlacement.EquallySpacedConnector\",\"uuid\":\"bceb85c7-25a5-44d0-bafc-eda31cc970da\"}],\"packageUris\":[\"http://schema.mathworks.com/mf0/Connector/R2020b\"],\"version\":\"1.0\"}"
      mask Display: disp("DC Motor")
  PID Controller : Subsystem
  PS-Simulink Converter1 : nesl_utility/PS-Simulink Converter  PhysicalDomain=network_engine_domain  SubClassName=ps_output  LeftPortType=input  RightPortType=output  PseudoPeriodic=off  Frequencies=[]  VectorFormat=inherit  Unit=inherit  AffineConversion=off
  PS-Simulink Converter2 : nesl_utility/PS-Simulink Converter  PhysicalDomain=network_engine_domain  SubClassName=ps_output  LeftPortType=input  RightPortType=output  PseudoPeriodic=off  Frequencies=[]  VectorFormat=inherit  Unit=inherit  AffineConversion=off
  Simulink-PS Converter : nesl_utility/Simulink-PS Converter  PhysicalDomain=network_engine_domain  SubClassName=ps_input  LeftPortType=input  RightPortType=output  PseudoPeriodic=off  Frequencies=[]  NoiseDistribution=none  NoiseParameters=[]  Unit=rad/s  AffineConversion=off  FilteringAndDerivatives=filter  SimscapeFilterOrder=1  InputFilterTimeConstant=0.001  UdotUserProvided=0
  Simulink-PS Converter1 : nesl_utility/Simulink-PS Converter  PhysicalDomain=network_engine_domain  SubClassName=ps_input  LeftPortType=input  RightPortType=output  PseudoPeriodic=off  Frequencies=[]  NoiseDistribution=none  NoiseParameters=[]  Unit=rad/s  AffineConversion=off  FilteringAndDerivatives=filter  SimscapeFilterOrder=1  InputFilterTimeConstant=0.001  UdotUserProvided=0
  Torque Joint1 : PMIOPort  Side=Right
  Torque Joint2 : PMIOPort  Port=2  Side=Right
  tag scope: motorTorque1=global, motorTorque2=global
  wires:
  PS-Simulink Converter1/1 -> [motorTorque2]
  PS-Simulink Converter2/1 -> [motorTorque1]
  dq1_sensor/1 -> Simulink-PS Converter/1
  dq2_sensor/1 -> Simulink-PS Converter1/1
  actuatorTorque1/1 -> Motor/2(actuatorTorque)
  actuatorTorque2/1 -> Motor1/2(actuatorTorque)
  PID Controller/1(VOLTAGE) -> Motor/1(Voltage)
  PID Controller/2(VOLTAGE2) -> Motor1/1(Voltage)
  connections:
  PS-Simulink Converter1/LConn1 -- Motor1/LConn1 -- Torque Joint2/RConn1
  Motor/RConn1 -- Simulink-PS Converter/RConn1
  Motor1/RConn1 -- Simulink-PS Converter1/RConn1
  Motor/LConn1 -- Torque Joint1/RConn1 -- PS-Simulink Converter2/LConn1

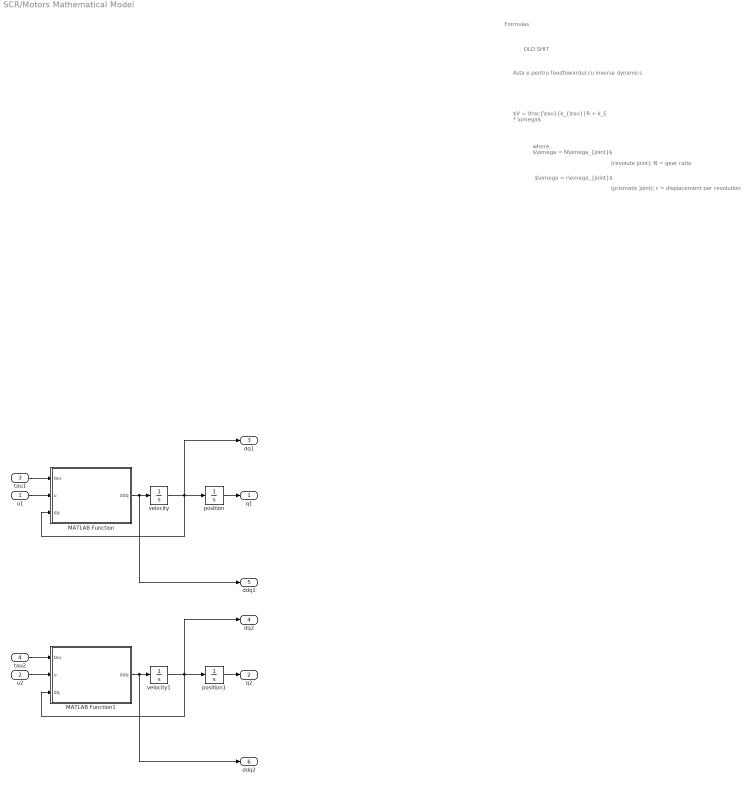
== system SCR/Motors Mathematical Model ==
  note: OLD SHIT
  note: Formulas
  note: $\omega = r\omega_{joint}$
  note: (revolute joint); N = gear ratio
  note: $\omega = N\omega_{joint}$
  note: where,
  note: $V = \frac{\tau}{k_{\tau}}R + k_E * \omega$
  note: (prismatic joint); r = displacement per revolution
  note: Asta e pentru feedfowardul cu inverse dynamics
  u1 : Inport
  u2 : Inport  Port=2
  tau1 : Inport  Port=3
  tau2 : Inport  Port=4
  MATLAB Function : MATLAB Function  TreatAsAtomicUnit=on
  MATLAB Function1 : MATLAB Function  TreatAsAtomicUnit=on
  position : Integrator
  position1 : Integrator
  velocity : Integrator
  velocity1 : Integrator
  q1 : Outport
  q2 : Outport  Port=2
  dq1 : Outport  Port=3
  dq2 : Outport  Port=4
  ddq1 : Outport  Port=5
  ddq2 : Outport  Port=6
  wires:
  tau1/1 -> MATLAB Function/1(tau)
  u1/1 -> MATLAB Function/2(u)
  MATLAB Function/1(ddq) -> ddq1/1, velocity/1
  velocity/1 -> dq1/1, MATLAB Function/3(dq), position/1
  position/1 -> q1/1
  position1/1 -> q2/1
  u2/1 -> MATLAB Function1/2(u)
  tau2/1 -> MATLAB Function1/1(tau)
  velocity1/1 -> dq2/1, MATLAB Function1/3(dq), position1/1
  MATLAB Function1/1(ddq) -> ddq2/1, velocity1/1
